simulink model "Final_RPO_Sim"  (R2024b)
settings: Solver=ode4  StartTime=0.0  StopTime=t_end  FixedStep=1  RelTol=1e-3
values from neighbouring files (symbols this model uses):
  A = [0       0    0     1     0   0 ... (first row only)    [rpo_setup.m]
  B = [zeros(3,3); eye(3)]    [rpo_setup.m]
  Gam = M(1:6,7:9)    [rpo_setup.m]
  H = [eye(3), zeros(3)]    [rpo_setup.m]
  K = lqr(A,B,Qw,Rw)    [rpo_setup.m]
  mu = 3.986004418e14    (= 398600441800000)    [rpo_setup.m]
  n = sqrt(mu/rt^3)    [rpo_setup.m]
  P0 = diag([P0pos^2*ones(1,3),             P0vel^2*ones(1,3)])    [rpo_setup.m]
  Phi = M(1:6,1:6)    [rpo_setup.m]
  Qd = (Qd + Qd')/2    [rpo_setup.m]
  R = sigma_z^2*eye(3)    [rpo_setup.m]
  rt = Re + 450e3    (= 6828137)    [rpo_setup.m]
  t_arrival = t_depart + t_tr    [rpo_setup.m]
  t_burn = 100    [rpo_setup.m]
  t_burn0 = 60    [rpo_setup.m]
  t_tr = 0.75*T    [rpo_setup.m]
  x0 = [0; -10000; 0; 0; 0; 0]    [rpo_setup.m]
  xh0 = x0 + chol(P0,'lower')*randn(6,1)    [rpo_setup.m]
settings Model: Creator=bhavy  LastModifiedBy=bhavy

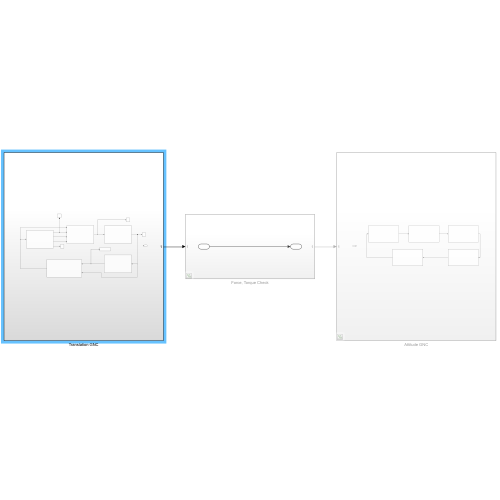
[thumbnail: Simulink's stored preview of the top-level diagram]
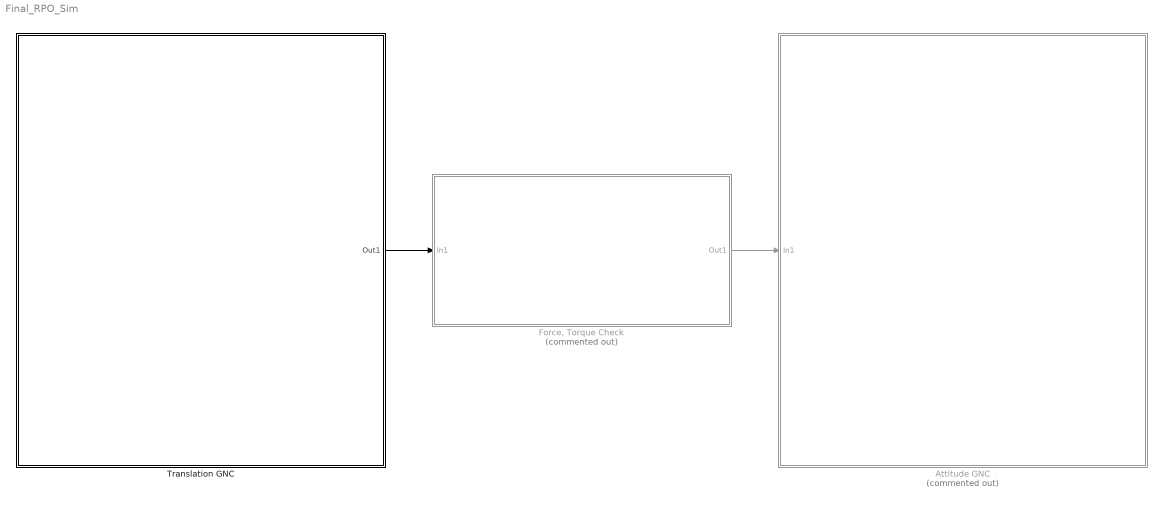
== system Final_RPO_Sim ==
  Attitude GNC : Subsystem  Commented=on
  "Force, Torque Check" : Subsystem  Commented=on
  Translation GNC : Subsystem
  wires:
  Translation GNC/1(Out1) -> "Force, Torque Check"/1(In1)
  "Force, Torque Check"/1(Out1) -> Attitude GNC/1(In1)

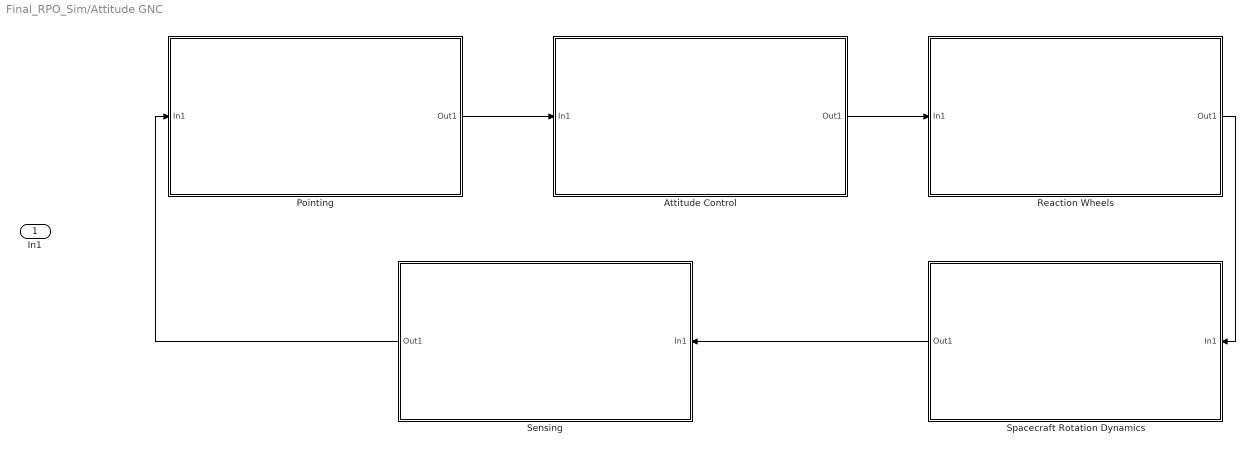
== system Final_RPO_Sim/Attitude GNC ==
  In1 : Inport
  Attitude Control : Subsystem
  Pointing : Subsystem
  Reaction Wheels : Subsystem
  Sensing : Subsystem
  Spacecraft Rotation Dynamics : Subsystem
  wires:
  Pointing/1(Out1) -> Attitude Control/1(In1)
  Attitude Control/1(Out1) -> Reaction Wheels/1(In1)
  Reaction Wheels/1(Out1) -> Spacecraft Rotation Dynamics/1(In1)
  Sensing/1(Out1) -> Pointing/1(In1)
  Spacecraft Rotation Dynamics/1(Out1) -> Sensing/1(In1)

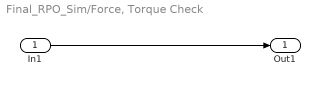
== system Final_RPO_Sim/Force, Torque Check ==
  In1 : Inport
  Out1 : Outport
  wires:
  In1/1 -> Out1/1

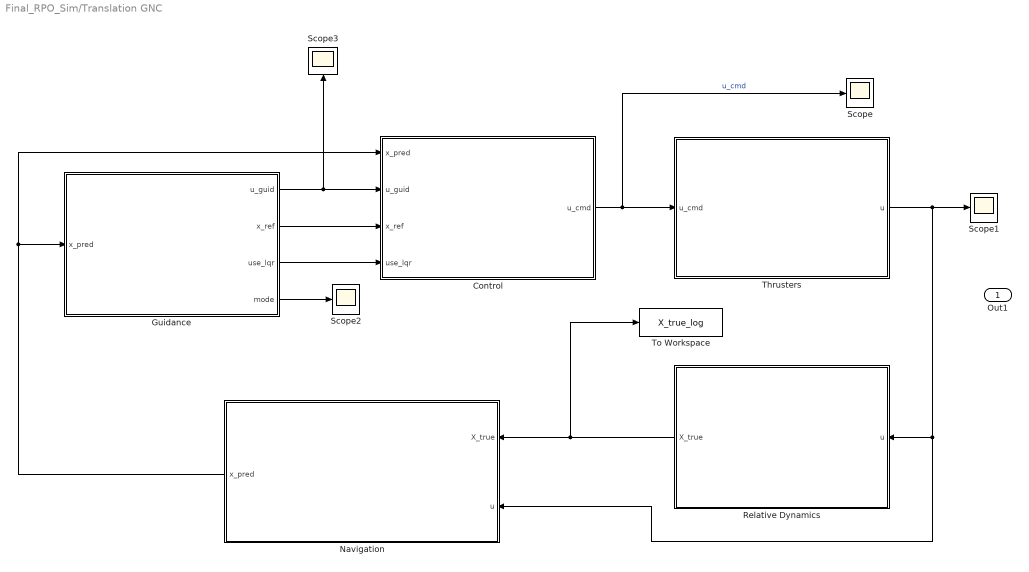
== system Final_RPO_Sim/Translation GNC ==
  Control : Subsystem
  Guidance : Subsystem
  Navigation : Subsystem
  Relative Dynamics : Subsystem
  Scope{,1..3} (4 alike) : Scope
  Thrusters : Subsystem
  To Workspace : ToWorkspace  VariableName=X_true_log  SaveFormat=Timeseries  SampleTime=-1
  Out1 : Outport
  wires:
  Control/1(u_cmd) -> Scope/1, Thrusters/1(u_cmd)  "u_cmd"
  Thrusters/1(u) -> Scope1/1, Relative Dynamics/1(u), Navigation/2(u)
  Relative Dynamics/1(X_true) -> To Workspace/1, Navigation/1(X_true)
  Navigation/1(x_pred) -> Control/1(x_pred), Guidance/1(x_pred)
  Guidance/3(use_lqr) -> Control/4(use_lqr)
  Guidance/2(x_ref) -> Control/3(x_ref)
  Guidance/1(u_guid) -> Scope3/1, Control/2(u_guid)
  Guidance/4(mode) -> Scope2/1

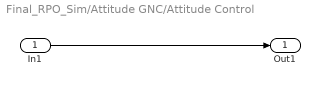
== system Final_RPO_Sim/Attitude GNC/Attitude Control ==
  In1 : Inport
  Out1 : Outport
  wires:
  In1/1 -> Out1/1

== system Final_RPO_Sim/Attitude GNC/Pointing ==
  In1 : Inport
  Out1 : Outport
  wires:
  In1/1 -> Out1/1

== system Final_RPO_Sim/Attitude GNC/Reaction Wheels ==
  In1 : Inport
  Out1 : Outport
  wires:
  In1/1 -> Out1/1

== system Final_RPO_Sim/Attitude GNC/Sensing ==
  In1 : Inport
  Out1 : Outport
  wires:
  In1/1 -> Out1/1

== system Final_RPO_Sim/Attitude GNC/Spacecraft Rotation Dynamics ==
  In1 : Inport
  Out1 : Outport
  wires:
  In1/1 -> Out1/1

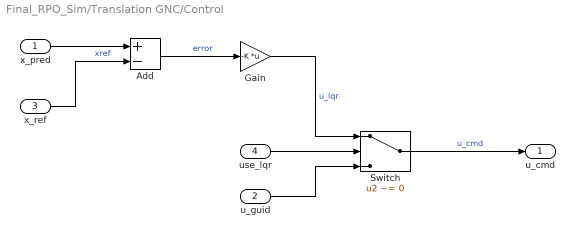
== system Final_RPO_Sim/Translation GNC/Control ==
  x_pred : Inport
  u_guid : Inport  Port=2
  x_ref : Inport  Port=3
  use_lqr : Inport  Port=4
  Add : Sum  Inputs=+-
  Gain : Gain  Gain=-K  Multiplication=Matrix(K*u)
  Switch : Switch  Criteria=u2 ~= 0  SaturateOnIntegerOverflow=off  InputSameDT=off
  u_cmd : Outport
  wires:
  x_ref/1 -> Add/2  "xref"
  Add/1 -> Gain/1  "error"
  Gain/1 -> Switch/1  "u_lqr"
  Switch/1 -> u_cmd/1  "u_cmd"
  use_lqr/1 -> Switch/2
  u_guid/1 -> Switch/3
  x_pred/1 -> Add/1

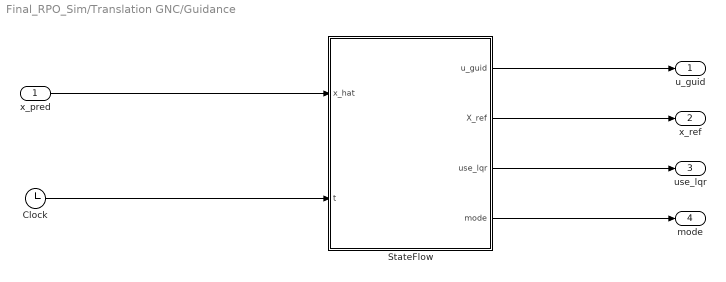
== system Final_RPO_Sim/Translation GNC/Guidance ==
  x_pred : Inport
  Clock : Clock
  StateFlow : Stateflow chart  TreatAsAtomicUnit=on
  u_guid : Outport
  x_ref : Outport  Port=2
  use_lqr : Outport  Port=3
  mode : Outport  Port=4
  wires:
  x_pred/1 -> StateFlow/1(x_hat)
  StateFlow/1(u_guid) -> u_guid/1
  StateFlow/2(X_ref) -> x_ref/1
  StateFlow/3(use_lqr) -> use_lqr/1
  StateFlow/4(mode) -> mode/1
  Clock/1 -> StateFlow/2(t)

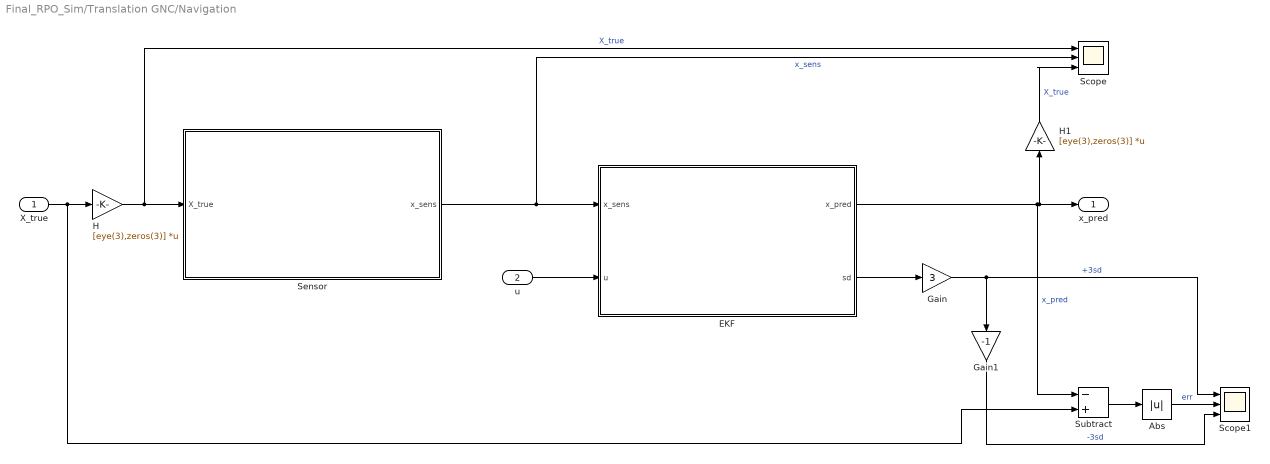
== system Final_RPO_Sim/Translation GNC/Navigation ==
  X_true : Inport
  u : Inport  Port=2
  Abs : Abs  SaturateOnIntegerOverflow=off
  EKF : Subsystem
  Gain : Gain  Gain=3
  Gain1 : Gain  Gain=-1
  H : Gain  Gain=[eye(3),zeros(3)]  Multiplication=Matrix(K*u)
  H1 : Gain  Gain=[eye(3),zeros(3)]  Multiplication=Matrix(K*u)
  Scope : Scope  NumInputPorts=3
  Scope1 : Scope  NumInputPorts=3
  Sensor : Subsystem
  Subtract : Sum  Inputs=-+
  x_pred : Outport
  wires:
  X_true/1 -> Subtract/2, H/1
  Sensor/1(x_sens) -> Scope/2, EKF/1(x_sens)  "x_sens"
  EKF/1(x_pred) -> x_pred/1, H1/1, Subtract/1  "x_pred"
  u/1 -> EKF/2(u)
  H/1 -> Scope/1, Sensor/1(X_true)  "X_true"
  Subtract/1 -> Abs/1
  Abs/1 -> Scope1/2  "err"
  EKF/2(sd) -> Gain/1
  Gain/1 -> Scope1/1, Gain1/1  "+3sd"
  Gain1/1 -> Scope1/3  "-3sd"
  H1/1 -> Scope/3  "X_true"

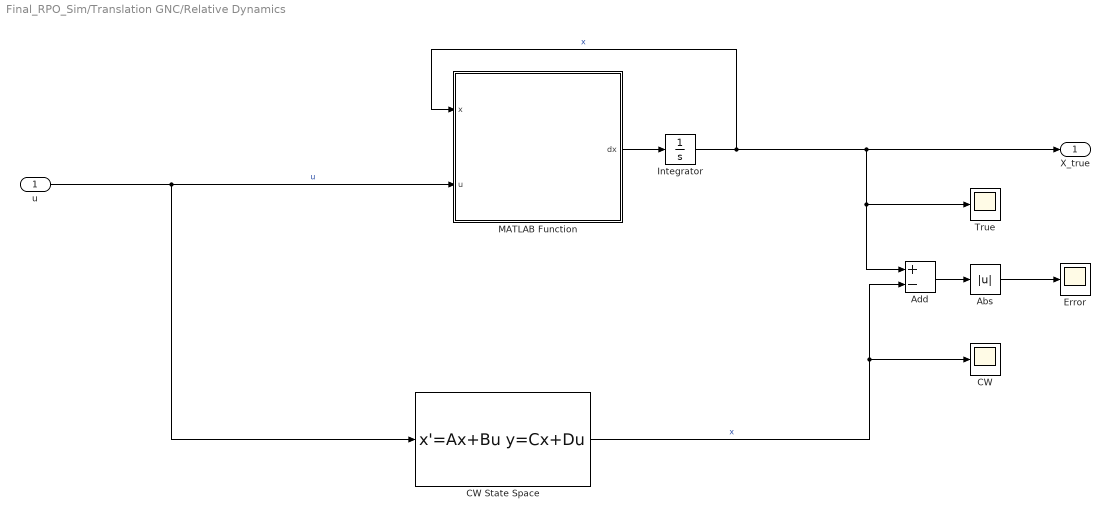
== system Final_RPO_Sim/Translation GNC/Relative Dynamics ==
  u : Inport
  Abs : Abs  SaturateOnIntegerOverflow=off
  Add : Sum  Inputs=+-
  CW : Scope
  CW State Space : StateSpace  A=A  B=B  C=eye(6)  D=zeros(6,3)  InitialCondition=x0
  Error : Scope
  Integrator : Integrator  InitialCondition=x0
  MATLAB Function : MATLAB Function  TreatAsAtomicUnit=on
  True : Scope
  X_true : Outport
  wires:
  u/1 -> CW State Space/1, MATLAB Function/2(u)  "u"
  MATLAB Function/1(dx) -> Integrator/1
  Integrator/1 -> MATLAB Function/1(x), X_true/1, Add/1, True/1  "x"
  CW State Space/1 -> Add/2, CW/1  "x"
  Add/1 -> Abs/1
  Abs/1 -> Error/1

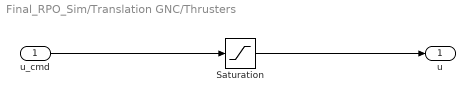
== system Final_RPO_Sim/Translation GNC/Thrusters ==
  u_cmd : Inport
  Saturation : Saturate  UpperLimit=0.01  LowerLimit=-0.01
  u : Outport
  wires:
  u_cmd/1 -> Saturation/1
  Saturation/1 -> u/1

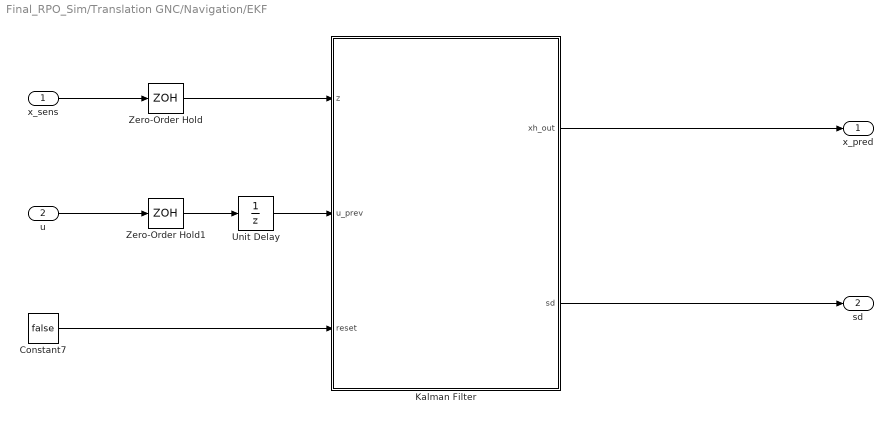
== system Final_RPO_Sim/Translation GNC/Navigation/EKF ==
  x_sens : Inport
  u : Inport  Port=2
  Constant7 : Constant  Value=false
  Kalman Filter : MATLAB Function  TreatAsAtomicUnit=on
  Unit Delay : UnitDelay  SampleTime=-1  HasFrameUpgradeWarning=on
  Zero-Order Hold : ZeroOrderHold
  Zero-Order Hold1 : ZeroOrderHold
  x_pred : Outport
  sd : Outport  Port=2
  wires:
  x_sens/1 -> Zero-Order Hold/1
  Kalman Filter/1(xh_out) -> x_pred/1
  Constant7/1 -> Kalman Filter/3(reset)
  Zero-Order Hold/1 -> Kalman Filter/1(z)
  u/1 -> Zero-Order Hold1/1
  Zero-Order Hold1/1 -> Unit Delay/1
  Unit Delay/1 -> Kalman Filter/2(u_prev)
  Kalman Filter/2(sd) -> sd/1

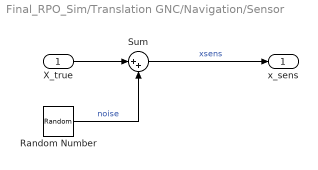
== system Final_RPO_Sim/Translation GNC/Navigation/Sensor ==
  X_true : Inport
  Random Number : RandomNumber  SampleTime=1
  Sum : Sum  Inputs=|++
  x_sens : Outport
  wires:
  X_true/1 -> Sum/1
  Random Number/1 -> Sum/2  "noise"
  Sum/1 -> x_sens/1  "xsens"

== matlab function Final_RPO_Sim/Translation GNC/Navigation/EKF/Kalman Filter ==
  data: z input; xh_out output; u_prev input; reset input boolean; sd output; Phi parameter; Gam parameter; Qd parameter; H parameter; R parameter; xh0 parameter; P0 parameter
function [xh_out, sd] = kf_step(z, u_prev, reset, Phi, Gam, Qd, H, R, xh0, P0)

persistent xh P initialized

if isempty(initialized)
    initialized = false;
    xh = zeros(6,1);
    P = zeros(6,6);
end

if ~initialized || reset
    xh = xh0;
    P = P0;
    initialized = true;

else
    % Prediction
    xh = Phi*xh + Gam*u_prev;

    % Covariance prediction
    P = Phi*P*Phi' + Qd;
end

% Innovation
y = z - H*xh;

% Innovation covariance
S = H*P*H' + R;

% Kalman gain
K = (P*H') / S;

% State correction
xh = xh + K*y;

% Covariance correction (Joseph form)
I_KH = eye(6) - K*H;
P = I_KH*P*I_KH' + K*R*K';

% Numerical symmetry
P = (P + P')/2;

xh_out = xh;
sd = sqrt(max(diag(P), 0));
end

== matlab function Final_RPO_Sim/Translation GNC/Relative Dynamics/MATLAB Function ==
  data: x input; u input; dx output; mu parameter; rt parameter; n parameter
function dx = nl_rel_dyn(x, u, mu, rt, n)

x = reshape(x, 6, 1);
u = reshape(u, 3, 1);

r = x(1:3);
v = x(4:6);

rc = sqrt((rt + r(1))^2 + r(2)^2 + r(3)^2);

a = zeros(3,1);

a(1) =  2*n*v(2) + n^2*r(1) - mu*(rt+r(1))/rc^3 + mu/rt^2 + u(1);
a(2) = -2*n*v(1) + n^2*r(2) - mu*r(2)/rc^3 + u(2);
a(3) = -mu*r(3)/rc^3 + u(3);

dx = [v; a];

end

== stateflow chart Final_RPO_Sim/Translation GNC/Guidance/StateFlow ==
  state Midcourse
    entry:
    dv_mid_cmd = calc_dv(x_hat, [0;-1000;0], t_arrival-t-t_burn/2, n);
    during:
    u_guid = dv_mid_cmd/t_burn;
    X_ref = [0;-1000;0;0;0;0];
    use_lqr = false;
    mode = 4;
  state Burn1
    entry:
    dv1_cmd = calc_dv(x_hat, [0;-1000;0], t_tr, n);
    during:
    u_guid = dv1_cmd/t_burn;
    X_ref = [0;-1000;0;0;0;0];
    use_lqr = false;
    mode = 2;
  state Coast_start
    during:
    u_guid = zeros(3,1);
    X_ref = [0;-1000;0;0;0;0];
    use_lqr = false;
    mode = 1;
  state Transfer
    during:
    u_guid = zeros(3,1);
    X_ref = [0;-1000;0;0;0;0];
    use_lqr = false;
    mode = 3;
  state Burn2
    entry:
    dv2_cmd = -x_hat(4:6);
    during:
    u_guid = dv2_cmd/t_burn;
    X_ref = [0;-1000;0;0;0;0];
    use_lqr = false;
    mode = 6;
  state Hold
    during:
    u_guid = zeros(3,1);
    X_ref = [0;-1000;0;0;0;0];
    use_lqr = true;
    mode = 7;
  state Transfer2
    during:
    u_guid = zeros(3,1);
    X_ref = [0;-1000;0;0;0;0];
    use_lqr = false;
    mode = 5;
  (default) -> (junction 38)
  Transfer -> Midcourse : [after(t_tr/2-t_burn,sec)]
  Coast_start -> Burn1 : [after(t_burn0,sec)]
  (junction 38) -> Coast_start
  Burn1 -> Transfer : [after(t_burn,sec)]
  Midcourse -> Transfer2 : [after(t_burn,sec)]
  Burn2 -> Hold : [after(t_burn,sec)]
  Transfer2 -> Burn2 : [after(t_tr/2-t_burn,sec)]
  data: x function_input; rf function_input; tf function_input; n function_input; dv function_output; x_hat input double size=[6 1]; u_guid output double size=[3 1]; X_ref output double size=[6 1]; use_lqr output boolean size=1; mode output double size=1; dv1_cmd local size=[3 1]; dv_mid_cmd local size=[3 1]; dv2_cmd local size=[3 1]; t_tr parameter; t input; t_burn parameter; t_burn0 parameter; t_arrival parameter; n parameter
  function dv = calc_dv(x, rf, tf, n):
    | function dv = calc_dv(x, rf, tf, n)
    | 
    | r0 = x(1:3);
    | v0 = x(4:6);
    | 
    | c = cos(n*tf);
    | s = sin(n*tf);
    | 
    | Prr = [4-3*c,       0, 0;
    |        6*(s-n*tf),  1, 0;
    |        0,           0, c];
    | 
    | Prv = [s/n,           2*(1-c)/n,       0;
    |        2*(c-1)/n,     (4*s-3*n*tf)/n, 0;
    |        0,             0,              s/n];
    | 
    | v_depart = Prv \ (rf - Prr*r0);
    | 
    | dv = v_depart - v0;
    | 
    | end
